simulink model "s_b4a4x32kf_54"  (R2018a)
settings: Solver=VariableStepDiscrete  StartTime=0.0  StopTime=10000  RelTol=1e-3
undefined symbols (not defined in the file): fft_stages, n_bits_ants, n_bits_xengs
libraries: xbsIndex_r4 x21235, casper_library_misc x37, casper_library_scopes x13, casper_library_delays x8, xbsReplacements_r4 x6, xps_library x4
(part 160 of 274)

== system s_b4a4x32kf_54/sys2/bf_pack_out0/Subsystem3/pipeline55 ==
  d : Inport
  Register0 : xbsIndex_r4/Register  init=0  rst=off  en=off  dbl_ovrd=off  block_type=register
      settings: SourceProductName=The database /home/jmanley/.matlab/R2018a/slblocks_master.db is locked, or a table in the database is locked. (database is locked)  block_version=11.4
  Register1 : xbsIndex_r4/Register  init=0  rst=off  en=off  dbl_ovrd=off  block_type=register
      settings: SourceProductName=The database /home/jmanley/.matlab/R2018a/slblocks_master.db is locked, or a table in the database is locked. (database is locked)  block_version=11.4
  q : Outport
  wires:
  Register0/1 -> Register1/1
  d/1 -> Register0/1
  Register1/1 -> q/1

== system s_b4a4x32kf_54/sys2/bf_pack_out0/Subsystem3/pipeline7 ==
  d : Inport
  Register0 : xbsIndex_r4/Register  init=0  rst=off  en=off  dbl_ovrd=off  block_type=register
      settings: SourceProductName=The database /home/jmanley/.matlab/R2018a/slblocks_master.db is locked, or a table in the database is locked. (database is locked)  block_version=11.4
  Register1 : xbsIndex_r4/Register  init=0  rst=off  en=off  dbl_ovrd=off  block_type=register
      settings: SourceProductName=The database /home/jmanley/.matlab/R2018a/slblocks_master.db is locked, or a table in the database is locked. (database is locked)  block_version=11.4
  q : Outport
  wires:
  Register0/1 -> Register1/1
  d/1 -> Register0/1
  Register1/1 -> q/1

== system s_b4a4x32kf_54/sys2/bf_pack_out0/data_fifo/bus_replicate ==
  in : Inport
  bussify : Subsystem  AncestorBlock=casper_library_flow_control/bus_create  mask(bus_create){inputNum=16}
      mask prompts: inputNum "Number of inputs:"
      mask init:
      | bus_create_init(gcb,...
      |     'inputNum', inputNum);
  out : Outport
  wires:
  in/1 -> bussify/1(in1), bussify/2(in2), bussify/3(in3), bussify/4(in4), bussify/5(in5), bussify/6(in6), bussify/7(in7), bussify/8(in8), bussify/9(in9), bussify/10(in10), bussify/11(in11), bussify/12(in12), bussify/13(in13), bussify/14(in14), bussify/15(in15), bussify/16(in16)
  bussify/1(bus_out) -> out/1

== system s_b4a4x32kf_54/sys2/bf_pack_out0/data_fifo/edge_detect ==
  in : Inport
  Delay : xbsIndex_r4/Delay  rst=off  infoeditControl=Selection of Reset will increase slice count due to use of real FFs and instead of SRLs  en=off  latency=1  reg_retiming=off  dbl_ovrd=off  block_type=delay
      settings: SourceProductName=The database /home/jmanley/.matlab/R2018a/slblocks_master.db is locked, or a table in the database is locked. (database is locked)  xl_area=[0, 0, 0, 0, 0, 0, 0]
  Inverter : xbsIndex_r4/Inverter  en=off  latency=0  dbl_ovrd=off  block_type=inv
      settings: SourceProductName=The database /home/jmanley/.matlab/R2018a/slblocks_master.db is locked, or a table in the database is locked. (database is locked)  xl_area=[0, 0, 0, 0, 0, 0, 0]
  edge_op : xbsIndex_r4/Logical  logical_function=AND  inputs=2  en=off  latency=0  precision=Full  arith_type=Unsigned  n_bits=8  bin_pt=2  align_bp=on  dbl_ovrd=off  block_type=logical
      settings: SourceProductName=The database /home/jmanley/.matlab/R2018a/slblocks_master.db is locked, or a table in the database is locked. (database is locked)  xl_area=[0, 0, 0, 0, 0, 0, 0]
  out : Outport
  wires:
  Inverter/1 -> edge_op/1
  edge_op/1 -> out/1
  in/1 -> Inverter/1, Delay/1
  Delay/1 -> edge_op/2

== system s_b4a4x32kf_54/sys2/bf_pack_out0/data_fifo/edge_detect1 ==
  in : Inport
  Delay : xbsIndex_r4/Delay  rst=off  infoeditControl=Selection of Reset will increase slice count due to use of real FFs and instead of SRLs  en=off  latency=1  reg_retiming=off  dbl_ovrd=off  block_type=delay
      settings: SourceProductName=The database /home/jmanley/.matlab/R2018a/slblocks_master.db is locked, or a table in the database is locked. (database is locked)  xl_area=[0, 0, 0, 0, 0, 0, 0]
  Inverter : xbsIndex_r4/Inverter  en=off  latency=0  dbl_ovrd=off  block_type=inv
      settings: SourceProductName=The database /home/jmanley/.matlab/R2018a/slblocks_master.db is locked, or a table in the database is locked. (database is locked)  xl_area=[0, 0, 0, 0, 0, 0, 0]
  edge_op : xbsIndex_r4/Logical  logical_function=AND  inputs=2  en=off  latency=0  precision=Full  arith_type=Unsigned  n_bits=8  bin_pt=2  align_bp=on  dbl_ovrd=off  block_type=logical
      settings: SourceProductName=The database /home/jmanley/.matlab/R2018a/slblocks_master.db is locked, or a table in the database is locked. (database is locked)  xl_area=[0, 0, 0, 0, 0, 0, 0]
  out : Outport
  wires:
  Inverter/1 -> edge_op/1
  edge_op/1 -> out/1
  in/1 -> Inverter/1, Delay/1
  Delay/1 -> edge_op/2

== system s_b4a4x32kf_54/sys2/bf_pack_out0/data_fifo/munge ==
  din : Inport
  join : Subsystem  AncestorBlock=casper_library_flow_control/bus_create  mask(bus_create){inputNum=16}
      mask prompts: inputNum "Number of inputs:"
      mask init:
      | bus_create_init(gcb,...
      |     'inputNum', inputNum);
  reinterpret : xbsIndex_r4/Reinterpret  force_arith_type=on  arith_type=Unsigned  force_bin_pt=on  bin_pt=0  block_type=reinterpret
      settings: SourceProductName=The database /home/jmanley/.matlab/R2018a/slblocks_master.db is locked, or a table in the database is locked. (database is locked)
  reinterpret_out : xbsIndex_r4/Reinterpret  force_arith_type=on  arith_type=Unsigned  force_bin_pt=on  bin_pt=0  block_type=reinterpret
      settings: SourceProductName=The database /home/jmanley/.matlab/R2018a/slblocks_master.db is locked, or a table in the database is locked. (database is locked)
  split : Subsystem  AncestorBlock=casper_library_flow_control/bus_expand  mask(bus_expand){mode=divisions of arbitrary size, outputNum=1, outputWidth=[16 16 16 16 16 16 16 16 16 16 16 16 16 16 16 16], outputBinaryPt=[0 0 0 0 0 0 0 0 0 0 0 0 0 0 0 0], outputArithmeticType=[0 0 0 0 0 0 0 0 0 0 0 0 0 0 0 0], show_format=off, outputToWorkspace=off, variablePrefix=out, outputToModelAsWell=on}
      mask prompts: outputNum "Number of outputs:"; outputWidth "Output width [msb ... lsb]:"; outputBinaryPt "Output binary point position [msb ... lsb]:"; outputArithmeticType "Output arithmetic type (ufix=0, fix=1, bool=2) [msb ... lsb]:"; show_format "Print format string?"; outputToWorkspace "Output to workspace?"; variablePrefix "Variable name prefix:"; outputToModelAsWell "Output to model as well?"
      mask help:
      | Expands a 'bus' made using a bus_create or Xilinx
      | concat block.
      | The input will be divided into the specified number
      | of outputs with the specified arithmetic types.
      | Divisions are made from most significant bit.
      mask init: same as s_b4a4x32kf_54/bus_expand
      settings: AttributesFormatString=16 outputs
      mask TypeOptions mode: divisions of equal size | divisions of arbitrary size
      mask Callback mode: bus_expand_callback();
      mask Callback outputWidth: bus_expand_callback();
      mask Callback outputToWorkspace: bus_expand_callback();
  dout : Outport
  wires:
  reinterpret_out/1 -> dout/1
  din/1 -> reinterpret/1
  reinterpret/1 -> split/1(bus_in)
  join/1(bus_out) -> reinterpret_out/1
  split/16(lsb_out1) -> join/1(in1)
  split/15(out2) -> join/2(in2)
  split/14(out3) -> join/3(in3)
  split/13(out4) -> join/4(in4)
  split/12(out5) -> join/5(in5)
  split/11(out6) -> join/6(in6)
  split/10(out7) -> join/7(in7)
  split/9(out8) -> join/8(in8)
  split/8(out9) -> join/9(in9)
  split/7(out10) -> join/10(in10)
  split/6(out11) -> join/11(in11)
  split/5(out12) -> join/12(in12)
  split/4(out13) -> join/13(in13)
  split/3(out14) -> join/14(in14)
  split/2(out15) -> join/15(in15)
  split/1(msb_out16) -> join/16(in16)

== system s_b4a4x32kf_54/sys2/bf_pack_out0/pack/edge_detect1 ==
  in : Inport
  Delay : xbsIndex_r4/Delay  rst=off  infoeditControl=Selection of Reset will increase slice count due to use of real FFs and instead of SRLs  en=off  latency=1  reg_retiming=off  dbl_ovrd=off  block_type=delay
      settings: SourceProductName=The database /home/jmanley/.matlab/R2018a/slblocks_master.db is locked, or a table in the database is locked. (database is locked)  xl_area=[0, 0, 0, 0, 0, 0, 0]
  Inverter : xbsIndex_r4/Inverter  en=off  latency=0  dbl_ovrd=off  block_type=inv
      settings: SourceProductName=The database /home/jmanley/.matlab/R2018a/slblocks_master.db is locked, or a table in the database is locked. (database is locked)  xl_area=[0, 0, 0, 0, 0, 0, 0]
  edge_op : xbsIndex_r4/Logical  logical_function=AND  inputs=2  en=off  latency=0  precision=Full  arith_type=Unsigned  n_bits=8  bin_pt=2  align_bp=on  dbl_ovrd=off  block_type=logical
      settings: SourceProductName=The database /home/jmanley/.matlab/R2018a/slblocks_master.db is locked, or a table in the database is locked. (database is locked)  xl_area=[0, 0, 0, 0, 0, 0, 0]
  out : Outport
  wires:
  Inverter/1 -> edge_op/1
  edge_op/1 -> out/1
  in/1 -> Inverter/1, Delay/1
  Delay/1 -> edge_op/2

== system s_b4a4x32kf_54/sys2/bf_pack_out0/pack/edge_detect3 ==
  in : Inport
  Delay : xbsIndex_r4/Delay  rst=off  infoeditControl=Selection of Reset will increase slice count due to use of real FFs and instead of SRLs  en=off  latency=1  reg_retiming=off  dbl_ovrd=off  block_type=delay
      settings: SourceProductName=The database /home/jmanley/.matlab/R2018a/slblocks_master.db is locked, or a table in the database is locked. (database is locked)  xl_area=[0, 0, 0, 0, 0, 0, 0]
  Inverter : xbsIndex_r4/Inverter  en=off  latency=0  dbl_ovrd=off  block_type=inv
      settings: SourceProductName=The database /home/jmanley/.matlab/R2018a/slblocks_master.db is locked, or a table in the database is locked. (database is locked)  xl_area=[0, 0, 0, 0, 0, 0, 0]
  edge_op : xbsIndex_r4/Logical  logical_function=NOR  inputs=2  en=off  latency=0  precision=Full  arith_type=Unsigned  n_bits=8  bin_pt=2  align_bp=on  dbl_ovrd=off  block_type=logical
      settings: SourceProductName=The database /home/jmanley/.matlab/R2018a/slblocks_master.db is locked, or a table in the database is locked. (database is locked)  xl_area=[0, 0, 0, 0, 0, 0, 0]
  out : Outport
  wires:
  Inverter/1 -> edge_op/1
  edge_op/1 -> out/1
  in/1 -> Inverter/1, Delay/1
  Delay/1 -> edge_op/2

== system s_b4a4x32kf_54/sys2/bf_pack_out1/Subsystem3/edge_detect ==
  in : Inport
  Delay : xbsIndex_r4/Delay  rst=off  infoeditControl=Selection of Reset will increase slice count due to use of real FFs and instead of SRLs  en=off  latency=1  reg_retiming=off  dbl_ovrd=off  block_type=delay
      settings: SourceProductName=The database /home/jmanley/.matlab/R2018a/slblocks_master.db is locked, or a table in the database is locked. (database is locked)  xl_area=[0, 0, 0, 0, 0, 0, 0]
  Inverter : xbsIndex_r4/Inverter  en=off  latency=0  dbl_ovrd=off  block_type=inv
      settings: SourceProductName=The database /home/jmanley/.matlab/R2018a/slblocks_master.db is locked, or a table in the database is locked. (database is locked)  xl_area=[0, 0, 0, 0, 0, 0, 0]
  edge_op : xbsIndex_r4/Logical  logical_function=NOR  inputs=2  en=off  latency=0  precision=Full  arith_type=Unsigned  n_bits=8  bin_pt=2  align_bp=on  dbl_ovrd=off  block_type=logical
      settings: SourceProductName=The database /home/jmanley/.matlab/R2018a/slblocks_master.db is locked, or a table in the database is locked. (database is locked)  xl_area=[0, 0, 0, 0, 0, 0, 0]
  out : Outport
  wires:
  Inverter/1 -> edge_op/1
  edge_op/1 -> out/1
  in/1 -> Inverter/1, Delay/1
  Delay/1 -> edge_op/2

== system s_b4a4x32kf_54/sys2/bf_pack_out1/Subsystem3/edge_detect1 ==
  in : Inport
  Delay : xbsIndex_r4/Delay  rst=off  infoeditControl=Selection of Reset will increase slice count due to use of real FFs and instead of SRLs  en=off  latency=1  reg_retiming=off  dbl_ovrd=off  block_type=delay
      settings: SourceProductName=The database /home/jmanley/.matlab/R2018a/slblocks_master.db is locked, or a table in the database is locked. (database is locked)  xl_area=[0, 0, 0, 0, 0, 0, 0]
  Inverter : xbsIndex_r4/Inverter  en=off  latency=0  dbl_ovrd=off  block_type=inv
      settings: SourceProductName=The database /home/jmanley/.matlab/R2018a/slblocks_master.db is locked, or a table in the database is locked. (database is locked)  xl_area=[0, 0, 0, 0, 0, 0, 0]
  edge_op : xbsIndex_r4/Logical  logical_function=NOR  inputs=2  en=off  latency=0  precision=Full  arith_type=Unsigned  n_bits=8  bin_pt=2  align_bp=on  dbl_ovrd=off  block_type=logical
      settings: SourceProductName=The database /home/jmanley/.matlab/R2018a/slblocks_master.db is locked, or a table in the database is locked. (database is locked)  xl_area=[0, 0, 0, 0, 0, 0, 0]
  out : Outport
  wires:
  Inverter/1 -> edge_op/1
  edge_op/1 -> out/1
  in/1 -> Inverter/1, Delay/1
  Delay/1 -> edge_op/2

== system s_b4a4x32kf_54/sys2/bf_pack_out1/Subsystem3/pipeline1 ==
  d : Inport
  Register0 : xbsIndex_r4/Register  init=0  rst=off  en=off  dbl_ovrd=off  block_type=register
      settings: SourceProductName=The database /home/jmanley/.matlab/R2018a/slblocks_master.db is locked, or a table in the database is locked. (database is locked)  block_version=11.4
  Register1 : xbsIndex_r4/Register  init=0  rst=off  en=off  dbl_ovrd=off  block_type=register
      settings: SourceProductName=The database /home/jmanley/.matlab/R2018a/slblocks_master.db is locked, or a table in the database is locked. (database is locked)  block_version=11.4
  q : Outport
  wires:
  Register0/1 -> Register1/1
  d/1 -> Register0/1
  Register1/1 -> q/1

== system s_b4a4x32kf_54/sys2/bf_pack_out1/Subsystem3/pipeline2 ==
  d : Inport
  Register0 : xbsIndex_r4/Register  init=0  rst=off  en=off  dbl_ovrd=off  block_type=register
      settings: SourceProductName=The database /home/jmanley/.matlab/R2018a/slblocks_master.db is locked, or a table in the database is locked. (database is locked)  block_version=11.4
  Register1 : xbsIndex_r4/Register  init=0  rst=off  en=off  dbl_ovrd=off  block_type=register
      settings: SourceProductName=The database /home/jmanley/.matlab/R2018a/slblocks_master.db is locked, or a table in the database is locked. (database is locked)  block_version=11.4
  q : Outport
  wires:
  Register0/1 -> Register1/1
  d/1 -> Register0/1
  Register1/1 -> q/1

== system s_b4a4x32kf_54/sys2/bf_pack_out1/Subsystem3/pipeline53 ==
  d : Inport
  Register0 : xbsIndex_r4/Register  init=0  rst=off  en=off  dbl_ovrd=off  block_type=register
      settings: SourceProductName=The database /home/jmanley/.matlab/R2018a/slblocks_master.db is locked, or a table in the database is locked. (database is locked)  block_version=11.4
  Register1 : xbsIndex_r4/Register  init=0  rst=off  en=off  dbl_ovrd=off  block_type=register
      settings: SourceProductName=The database /home/jmanley/.matlab/R2018a/slblocks_master.db is locked, or a table in the database is locked. (database is locked)  block_version=11.4
  q : Outport
  wires:
  Register0/1 -> Register1/1
  d/1 -> Register0/1
  Register1/1 -> q/1

== system s_b4a4x32kf_54/sys2/bf_pack_out1/Subsystem3/pipeline54 ==
  d : Inport
  Register0 : xbsIndex_r4/Register  init=0  rst=off  en=off  dbl_ovrd=off  block_type=register
      settings: SourceProductName=The database /home/jmanley/.matlab/R2018a/slblocks_master.db is locked, or a table in the database is locked. (database is locked)  block_version=11.4
  Register1 : xbsIndex_r4/Register  init=0  rst=off  en=off  dbl_ovrd=off  block_type=register
      settings: SourceProductName=The database /home/jmanley/.matlab/R2018a/slblocks_master.db is locked, or a table in the database is locked. (database is locked)  block_version=11.4
  q : Outport
  wires:
  Register0/1 -> Register1/1
  d/1 -> Register0/1
  Register1/1 -> q/1

== system s_b4a4x32kf_54/sys2/bf_pack_out1/Subsystem3/pipeline55 ==
  d : Inport
  Register0 : xbsIndex_r4/Register  init=0  rst=off  en=off  dbl_ovrd=off  block_type=register
      settings: SourceProductName=The database /home/jmanley/.matlab/R2018a/slblocks_master.db is locked, or a table in the database is locked. (database is locked)  block_version=11.4
  Register1 : xbsIndex_r4/Register  init=0  rst=off  en=off  dbl_ovrd=off  block_type=register
      settings: SourceProductName=The database /home/jmanley/.matlab/R2018a/slblocks_master.db is locked, or a table in the database is locked. (database is locked)  block_version=11.4
  q : Outport
  wires:
  Register0/1 -> Register1/1
  d/1 -> Register0/1
  Register1/1 -> q/1

== system s_b4a4x32kf_54/sys2/bf_pack_out1/Subsystem3/pipeline7 ==
  d : Inport
  Register0 : xbsIndex_r4/Register  init=0  rst=off  en=off  dbl_ovrd=off  block_type=register
      settings: SourceProductName=The database /home/jmanley/.matlab/R2018a/slblocks_master.db is locked, or a table in the database is locked. (database is locked)  block_version=11.4
  Register1 : xbsIndex_r4/Register  init=0  rst=off  en=off  dbl_ovrd=off  block_type=register
      settings: SourceProductName=The database /home/jmanley/.matlab/R2018a/slblocks_master.db is locked, or a table in the database is locked. (database is locked)  block_version=11.4
  q : Outport
  wires:
  Register0/1 -> Register1/1
  d/1 -> Register0/1
  Register1/1 -> q/1

== system s_b4a4x32kf_54/sys2/bf_pack_out1/data_fifo/bus_replicate ==
  in : Inport
  bussify : Subsystem  AncestorBlock=casper_library_flow_control/bus_create  mask(bus_create){inputNum=16}
      mask prompts: inputNum "Number of inputs:"
      mask init:
      | bus_create_init(gcb,...
      |     'inputNum', inputNum);
  out : Outport
  wires:
  in/1 -> bussify/1(in1), bussify/2(in2), bussify/3(in3), bussify/4(in4), bussify/5(in5), bussify/6(in6), bussify/7(in7), bussify/8(in8), bussify/9(in9), bussify/10(in10), bussify/11(in11), bussify/12(in12), bussify/13(in13), bussify/14(in14), bussify/15(in15), bussify/16(in16)
  bussify/1(bus_out) -> out/1

== system s_b4a4x32kf_54/sys2/bf_pack_out1/data_fifo/edge_detect ==
  in : Inport
  Delay : xbsIndex_r4/Delay  rst=off  infoeditControl=Selection of Reset will increase slice count due to use of real FFs and instead of SRLs  en=off  latency=1  reg_retiming=off  dbl_ovrd=off  block_type=delay
      settings: SourceProductName=The database /home/jmanley/.matlab/R2018a/slblocks_master.db is locked, or a table in the database is locked. (database is locked)  xl_area=[0, 0, 0, 0, 0, 0, 0]
  Inverter : xbsIndex_r4/Inverter  en=off  latency=0  dbl_ovrd=off  block_type=inv
      settings: SourceProductName=The database /home/jmanley/.matlab/R2018a/slblocks_master.db is locked, or a table in the database is locked. (database is locked)  xl_area=[0, 0, 0, 0, 0, 0, 0]
  edge_op : xbsIndex_r4/Logical  logical_function=AND  inputs=2  en=off  latency=0  precision=Full  arith_type=Unsigned  n_bits=8  bin_pt=2  align_bp=on  dbl_ovrd=off  block_type=logical
      settings: SourceProductName=The database /home/jmanley/.matlab/R2018a/slblocks_master.db is locked, or a table in the database is locked. (database is locked)  xl_area=[0, 0, 0, 0, 0, 0, 0]
  out : Outport
  wires:
  Inverter/1 -> edge_op/1
  edge_op/1 -> out/1
  in/1 -> Inverter/1, Delay/1
  Delay/1 -> edge_op/2

== system s_b4a4x32kf_54/sys2/bf_pack_out1/data_fifo/edge_detect1 ==
  in : Inport
  Delay : xbsIndex_r4/Delay  rst=off  infoeditControl=Selection of Reset will increase slice count due to use of real FFs and instead of SRLs  en=off  latency=1  reg_retiming=off  dbl_ovrd=off  block_type=delay
      settings: SourceProductName=The database /home/jmanley/.matlab/R2018a/slblocks_master.db is locked, or a table in the database is locked. (database is locked)  xl_area=[0, 0, 0, 0, 0, 0, 0]
  Inverter : xbsIndex_r4/Inverter  en=off  latency=0  dbl_ovrd=off  block_type=inv
      settings: SourceProductName=The database /home/jmanley/.matlab/R2018a/slblocks_master.db is locked, or a table in the database is locked. (database is locked)  xl_area=[0, 0, 0, 0, 0, 0, 0]
  edge_op : xbsIndex_r4/Logical  logical_function=AND  inputs=2  en=off  latency=0  precision=Full  arith_type=Unsigned  n_bits=8  bin_pt=2  align_bp=on  dbl_ovrd=off  block_type=logical
      settings: SourceProductName=The database /home/jmanley/.matlab/R2018a/slblocks_master.db is locked, or a table in the database is locked. (database is locked)  xl_area=[0, 0, 0, 0, 0, 0, 0]
  out : Outport
  wires:
  Inverter/1 -> edge_op/1
  edge_op/1 -> out/1
  in/1 -> Inverter/1, Delay/1
  Delay/1 -> edge_op/2

== system s_b4a4x32kf_54/sys2/bf_pack_out1/data_fifo/munge ==
  din : Inport
  join : Subsystem  AncestorBlock=casper_library_flow_control/bus_create  mask(bus_create){inputNum=16}
      mask prompts: inputNum "Number of inputs:"
      mask init:
      | bus_create_init(gcb,...
      |     'inputNum', inputNum);
  reinterpret : xbsIndex_r4/Reinterpret  force_arith_type=on  arith_type=Unsigned  force_bin_pt=on  bin_pt=0  block_type=reinterpret
      settings: SourceProductName=The database /home/jmanley/.matlab/R2018a/slblocks_master.db is locked, or a table in the database is locked. (database is locked)
  reinterpret_out : xbsIndex_r4/Reinterpret  force_arith_type=on  arith_type=Unsigned  force_bin_pt=on  bin_pt=0  block_type=reinterpret
      settings: SourceProductName=The database /home/jmanley/.matlab/R2018a/slblocks_master.db is locked, or a table in the database is locked. (database is locked)
  split : Subsystem  AncestorBlock=casper_library_flow_control/bus_expand  mask(bus_expand){mode=divisions of arbitrary size, outputNum=1, outputWidth=[16 16 16 16 16 16 16 16 16 16 16 16 16 16 16 16], outputBinaryPt=[0 0 0 0 0 0 0 0 0 0 0 0 0 0 0 0], outputArithmeticType=[0 0 0 0 0 0 0 0 0 0 0 0 0 0 0 0], show_format=off, outputToWorkspace=off, variablePrefix=out, outputToModelAsWell=on}
      mask prompts: outputNum "Number of outputs:"; outputWidth "Output width [msb ... lsb]:"; outputBinaryPt "Output binary point position [msb ... lsb]:"; outputArithmeticType "Output arithmetic type (ufix=0, fix=1, bool=2) [msb ... lsb]:"; show_format "Print format string?"; outputToWorkspace "Output to workspace?"; variablePrefix "Variable name prefix:"; outputToModelAsWell "Output to model as well?"
      mask help:
      | Expands a 'bus' made using a bus_create or Xilinx
      | concat block.
      | The input will be divided into the specified number
      | of outputs with the specified arithmetic types.
      | Divisions are made from most significant bit.
      mask init: same as s_b4a4x32kf_54/bus_expand
      settings: AttributesFormatString=16 outputs
      mask TypeOptions mode: divisions of equal size | divisions of arbitrary size
      mask Callback mode: bus_expand_callback();
      mask Callback outputWidth: bus_expand_callback();
      mask Callback outputToWorkspace: bus_expand_callback();
  dout : Outport
  wires:
  reinterpret_out/1 -> dout/1
  din/1 -> reinterpret/1
  reinterpret/1 -> split/1(bus_in)
  join/1(bus_out) -> reinterpret_out/1
  split/16(lsb_out1) -> join/1(in1)
  split/15(out2) -> join/2(in2)
  split/14(out3) -> join/3(in3)
  split/13(out4) -> join/4(in4)
  split/12(out5) -> join/5(in5)
  split/11(out6) -> join/6(in6)
  split/10(out7) -> join/7(in7)
  split/9(out8) -> join/8(in8)
  split/8(out9) -> join/9(in9)
  split/7(out10) -> join/10(in10)
  split/6(out11) -> join/11(in11)
  split/5(out12) -> join/12(in12)
  split/4(out13) -> join/13(in13)
  split/3(out14) -> join/14(in14)
  split/2(out15) -> join/15(in15)
  split/1(msb_out16) -> join/16(in16)

== system s_b4a4x32kf_54/sys2/bf_pack_out1/pack/edge_detect1 ==
  in : Inport
  Delay : xbsIndex_r4/Delay  rst=off  infoeditControl=Selection of Reset will increase slice count due to use of real FFs and instead of SRLs  en=off  latency=1  reg_retiming=off  dbl_ovrd=off  block_type=delay
      settings: SourceProductName=The database /home/jmanley/.matlab/R2018a/slblocks_master.db is locked, or a table in the database is locked. (database is locked)  xl_area=[0, 0, 0, 0, 0, 0, 0]
  Inverter : xbsIndex_r4/Inverter  en=off  latency=0  dbl_ovrd=off  block_type=inv
      settings: SourceProductName=The database /home/jmanley/.matlab/R2018a/slblocks_master.db is locked, or a table in the database is locked. (database is locked)  xl_area=[0, 0, 0, 0, 0, 0, 0]
  edge_op : xbsIndex_r4/Logical  logical_function=AND  inputs=2  en=off  latency=0  precision=Full  arith_type=Unsigned  n_bits=8  bin_pt=2  align_bp=on  dbl_ovrd=off  block_type=logical
      settings: SourceProductName=The database /home/jmanley/.matlab/R2018a/slblocks_master.db is locked, or a table in the database is locked. (database is locked)  xl_area=[0, 0, 0, 0, 0, 0, 0]
  out : Outport
  wires:
  Inverter/1 -> edge_op/1
  edge_op/1 -> out/1
  in/1 -> Inverter/1, Delay/1
  Delay/1 -> edge_op/2

== system s_b4a4x32kf_54/sys2/bf_pack_out1/pack/edge_detect3 ==
  in : Inport
  Delay : xbsIndex_r4/Delay  rst=off  infoeditControl=Selection of Reset will increase slice count due to use of real FFs and instead of SRLs  en=off  latency=1  reg_retiming=off  dbl_ovrd=off  block_type=delay
      settings: SourceProductName=The database /home/jmanley/.matlab/R2018a/slblocks_master.db is locked, or a table in the database is locked. (database is locked)  xl_area=[0, 0, 0, 0, 0, 0, 0]
  Inverter : xbsIndex_r4/Inverter  en=off  latency=0  dbl_ovrd=off  block_type=inv
      settings: SourceProductName=The database /home/jmanley/.matlab/R2018a/slblocks_master.db is locked, or a table in the database is locked. (database is locked)  xl_area=[0, 0, 0, 0, 0, 0, 0]
  edge_op : xbsIndex_r4/Logical  logical_function=NOR  inputs=2  en=off  latency=0  precision=Full  arith_type=Unsigned  n_bits=8  bin_pt=2  align_bp=on  dbl_ovrd=off  block_type=logical
      settings: SourceProductName=The database /home/jmanley/.matlab/R2018a/slblocks_master.db is locked, or a table in the database is locked. (database is locked)  xl_area=[0, 0, 0, 0, 0, 0, 0]
  out : Outport
  wires:
  Inverter/1 -> edge_op/1
  edge_op/1 -> out/1
  in/1 -> Inverter/1, Delay/1
  Delay/1 -> edge_op/2

== system s_b4a4x32kf_54/sys2/pkt_reord/bus_replicate/bussify ==
  in1 : Inport
  reinterpret1 : xbsIndex_r4/Reinterpret  force_arith_type=on  arith_type=Unsigned  force_bin_pt=on  bin_pt=0  block_type=reinterpret
      settings: SourceProductName=The database /home/jmanley/.matlab/R2018a/slblocks_master.db is locked, or a table in the database is locked. (database is locked)  infoedit="Changes signal type without altering the binary representation.   You can changed the signal between signed and unsigned, and relocate the binary point.<br><br>Hardware notes: In hardware this block costs nothing.<br><br>Example:  Suppose the input is 6 bits wide, signed, with 2 fractional bits, and the output is forced to unsigned with 0 fractional bits.  Then an input of -2.0 (1110.00 in binary 2's complement) becomes an output of 56 (111000 in binary)."
  bus_out : Outport
  wires:
  in1/1 -> reinterpret1/1
  reinterpret1/1 -> bus_out/1

== system s_b4a4x32kf_54/sys2/pkt_reord/input_control/adder_tree ==
  sync : Inport
  din1 : Inport  Port=2
  din2 : Inport  Port=3
  din3 : Inport  Port=4
  addr1 : xbsIndex_r4/AddSub  mode=Addition  use_carryin=off  use_carryout=off  en=off  latency=2  precision=Full  arith_type=Unsigned  n_bits=16  bin_pt=14  quantization=Truncate  overflow=Wrap  use_behavioral_HDL=off  hw_selection=Fabric  pipelined=on  use_rpm=on  dbl_ovrd=off  block_type=addsub
      settings: SourceProductName=The database /home/jmanley/.matlab/R2018a/slblocks_master.db is locked, or a table in the database is locked. (database is locked)
  addr3 : xbsIndex_r4/AddSub  mode=Addition  use_carryin=off  use_carryout=off  en=off  latency=2  precision=Full  arith_type=Unsigned  n_bits=16  bin_pt=14  quantization=Truncate  overflow=Wrap  use_behavioral_HDL=off  hw_selection=Fabric  pipelined=on  use_rpm=on  dbl_ovrd=off  block_type=addsub
      settings: SourceProductName=The database /home/jmanley/.matlab/R2018a/slblocks_master.db is locked, or a table in the database is locked. (database is locked)
  dly2 : xbsIndex_r4/Delay  rst=off  infoeditControl=Selection of Reset will increase slice count due to use of real FFs and instead of SRLs  en=off  latency=2  reg_retiming=on  dbl_ovrd=off  block_type=delay
      settings: SourceProductName=The database /home/jmanley/.matlab/R2018a/slblocks_master.db is locked, or a table in the database is locked. (database is locked)
  sync_delay : xbsIndex_r4/Delay  rst=off  infoeditControl=Selection of Reset will increase slice count due to use of real FFs and instead of SRLs  en=off  latency=4  reg_retiming=on  dbl_ovrd=off  block_type=delay
      settings: SourceProductName=The database /home/jmanley/.matlab/R2018a/slblocks_master.db is locked, or a table in the database is locked. (database is locked)  block_version=11.4
  sync_out : Outport
  dout : Outport  Port=2
  wires:
  sync/1 -> sync_delay/1
  sync_delay/1 -> sync_out/1
  din1/1 -> addr1/1
  din2/1 -> addr1/2
  din3/1 -> dly2/1
  addr1/1 -> addr3/1
  dly2/1 -> addr3/2
  addr3/1 -> dout/1

== system s_b4a4x32kf_54/sys2/pkt_reord/input_control/mcnt_thresh ==
  note: we record if this is the first timestamp.
      | If it is we capture it even if out of bounds
  note: capture any new mcnts which
      | are within (1/2 buffer - 1)
      | of the previous mcnt.
      | This prevents locking onto
      | bad mcnts
  note: timeout of a bad
      | master count
      | in ~2^20 clocks
  mcnt : Inport
  en : Inport  Port=2
  AddSub : xbsIndex_r4/AddSub  mode=Addition  use_carryin=off  use_carryout=off  en=off  latency=2  precision=User Defined  arith_type=Unsigned  n_bits=n_bits_timestamp + (chan_bits-xeng_bits)  bin_pt=0  quantization=Truncate  overflow=Wrap  use_behavioral_HDL=on  hw_selection=Fabric  pipelined=off  dbl_ovrd=off  block_type=addsub
      settings: SourceProductName=The database /home/jmanley/.matlab/R2018a/slblocks_master.db is locked, or a table in the database is locked. (database is locked)
  Constant1 : xbsIndex_r4/Constant  const=(2^(window_bits - 2)) + 1  gui_display_data_type=Fixed-point  arith_type=Unsigned  n_bits=window_bits  bin_pt=0  preci_type=Single  exp_width=8  frac_width=24  explicit_period=on  period=1  equ=P=C  opselect=C  inp2=PCIN>>17  opr=+  inp1=P  carry=CIN  dbl_ovrd=off  block_type=constant
      settings: SourceProductName=The database /home/jmanley/.matlab/R2018a/slblocks_master.db is locked, or a table in the database is locked. (database is locked)
  Counter : xbsIndex_r4/Counter  cnt_type=Free Running  cnt_to=Inf  operation=Up  start_count=0  cnt_by_val=1  arith_type=Unsigned  n_bits=21  bin_pt=0  load_pin=off  rst=on  en=off  explicit_period=on  period=1  use_behavioral_HDL=off  implementation=Fabric  use_rpm=on  dbl_ovrd=off  block_type=counter
      settings: SourceProductName=The database /home/jmanley/.matlab/R2018a/slblocks_master.db is locked, or a table in the database is locked. (database is locked)  xl_area=[0, 0, 0, 0, 0, 0, 0]
  Delay : xbsIndex_r4/Delay  rst=off  infoeditControl=Selection of Reset will increase slice count due to use of real FFs and instead of SRLs  en=off  latency=2  reg_retiming=on  dbl_ovrd=off  block_type=delay
      settings: SourceProductName=The database /home/jmanley/.matlab/R2018a/slblocks_master.db is locked, or a table in the database is locked. (database is locked)  xl_area=[0, 0, 0, 0, 0, 0, 0]
  Delay1 : xbsIndex_r4/Delay  rst=off  infoeditControl=Selection of Reset will increase slice count due to use of real FFs and instead of SRLs  en=off  latency=1  reg_retiming=on  dbl_ovrd=off  block_type=delay
      settings: SourceProductName=The database /home/jmanley/.matlab/R2018a/slblocks_master.db is locked, or a table in the database is locked. (database is locked)  xl_area=[0, 0, 0, 0, 0, 0, 0]
  Gateway Out{,1..6} (7 alike) : xbsIndex_r4/Gateway Out  inherit_from_input=off  hdl_port=on  rows=1  columns=1  UseAsDAC=off  DACChannel='1'  interface=None  automatic_assignment=on  address_offset=hex2dec('00')  intf_name=''  intf_description=''  timing_constraint=None  locs_specified=off  LOCs={}  io_standard={}  block_type=gatewayout
      settings: SourceProductName=The database /home/jmanley/.matlab/R2018a/slblocks_master.db is locked, or a table in the database is locked. (database is locked)
  Inverter : xbsIndex_r4/Inverter  en=off  latency=0  dbl_ovrd=off  block_type=inv
      settings: SourceProductName=The database /home/jmanley/.matlab/R2018a/slblocks_master.db is locked, or a table in the database is locked. (database is locked)
  Logical : xbsIndex_r4/Logical  logical_function=AND  inputs=2  en=off  latency=0  precision=Full  arith_type=Unsigned  n_bits=8  bin_pt=2  align_bp=on  dbl_ovrd=off  block_type=logical
      settings: SourceProductName=The database /home/jmanley/.matlab/R2018a/slblocks_master.db is locked, or a table in the database is locked. (database is locked)  xl_area=[0, 0, 0, 0, 0, 0, 0]
  Logical1 : xbsIndex_r4/Logical  logical_function=OR  inputs=3  en=off  latency=0  precision=Full  arith_type=Unsigned  n_bits=8  bin_pt=2  align_bp=on  dbl_ovrd=off  block_type=logical
      settings: SourceProductName=The database /home/jmanley/.matlab/R2018a/slblocks_master.db is locked, or a table in the database is locked. (database is locked)  xl_area=[0, 0, 0, 0, 0, 0, 0]
  Register : xbsIndex_r4/Delay  rst=off  infoeditControl=Selection of Reset will increase slice count due to use of real FFs and instead of SRLs  en=on  latency=1  reg_retiming=on  dbl_ovrd=off  block_type=delay
      settings: SourceProductName=The database /home/jmanley/.matlab/R2018a/slblocks_master.db is locked, or a table in the database is locked. (database is locked)
  Relational : xbsIndex_r4/Relational  mode=a>b  op_type=Bool  en=off  latency=1  dbl_ovrd=off  block_type=relational
      settings: SourceProductName=The database /home/jmanley/.matlab/R2018a/slblocks_master.db is locked, or a table in the database is locked. (database is locked)  xl_area=[0, 0, 0, 0, 0, 0, 0]  block_version=10.1.3
  Relational1 : xbsIndex_r4/Relational  mode=a<=b  op_type=Bool  en=off  latency=1  dbl_ovrd=off  block_type=relational
      settings: SourceProductName=The database /home/jmanley/.matlab/R2018a/slblocks_master.db is locked, or a table in the database is locked. (database is locked)  xl_area=[0, 0, 0, 0, 0, 0, 0]  block_version=10.1.3
  Scope1 : Scope  NumInputPorts=7
  Slice : xbsIndex_r4/Slice  nbits=1  boolean_output=on  mode=Upper Bit Location + Width  bit1=0  base1=MSB of Input  bit0=0  base0=LSB of Input  dbl_ovrd=off  block_type=slice
      settings: SourceProductName=The database /home/jmanley/.matlab/R2018a/slblocks_master.db is locked, or a table in the database is locked. (database is locked)  infoedit="Extracts a given range of bits from each input sample and presents it at the output.  The output type is ordinarily unsigned with binary point at zero, but can be Boolean when the slice is one bit wide.<P><P>Hardware notes: In hardware this block costs nothing."  block_version=10.1.3
  edge_detect : Subsystem  mask(edge_detect){edge=Rising, polarity=Active High, x_in=[0 0.08 0.08 0.16 0.16 0.24 0.24 0.32 0.32 0.4], y_in=[-1 -1  1  1  1  1  1  1  1  1], x_out=[0.6 0.68 0.68 0.76 0.76 0.84 0.84 0.92 0.92 1], y_out=[-1 -1  1  1 -1 -1 -1 -1 -1 -1]}
      mask prompts: edge "Edge Type"; polarity "Output Polarity"; x_in "Input X Positions"; y_in "Input Y Positions"; x_out "Output X Positions"; y_out "Output Y Positions"
      mask help: Output is active for one-cycle after each edge of the specified type (i.e. rising, falling or both).
      mask init: same as s_b4a4x32kf_54/edge_detect
      settings: AttributesFormatString=|
      | rising edges
      | active high
      mask Help: Output is active for one-cycle after each edge of the specified type (i.e. rising, falling, or both).  Latency is zero.
      mask TypeOptions edge: Rising | Falling | Both
      mask TypeOptions polarity: Active High | Active Low
      mask Display:
      | plot(x_in_num,0.5+y_in_num*0.2);
      | plot(x_out_num,0.5+y_out_num*0.2);
  not_first : xbsIndex_r4/Delay  rst=off  infoeditControl=Selection of Reset will increase slice count due to use of real FFs and instead of SRLs  en=on  latency=1  reg_retiming=on  dbl_ovrd=off  block_type=delay
      settings: SourceProductName=The database /home/jmanley/.matlab/R2018a/slblocks_master.db is locked, or a table in the database is locked. (database is locked)
  maxcnt : Outport
  mcnt_timeout : Outport  Port=2
  wires:
  Relational1/1 -> Logical/2
  mcnt/1 -> Relational1/1, Relational/1, Gateway Out/1, Delay1/1
  Slice/1 -> edge_detect/1(in), Logical1/1
  Logical1/1 -> Counter/1, Register/2, Gateway Out4/1
  Logical/1 -> Logical1/2, Gateway Out2/1
  Counter/1 -> Gateway Out1/1, Slice/1
  Relational/1 -> Logical/1
  Register/1 -> AddSub/1, maxcnt/1, Gateway Out5/1, Delay/1
  AddSub/1 -> Gateway Out6/1, Relational1/2
  en/1 -> not_first/1, not_first/2
  Inverter/1 -> Gateway Out3/1, Logical1/3
  Delay1/1 -> Register/1
  Gateway Out/1 -> Scope1/1
  Gateway Out1/1 -> Scope1/2
  Gateway Out2/1 -> Scope1/3
  Gateway Out3/1 -> Scope1/4
  Gateway Out4/1 -> Scope1/5
  Gateway Out5/1 -> Scope1/6
  Gateway Out6/1 -> Scope1/7
  Delay/1 -> Relational/2
  not_first/1 -> Inverter/1
  Constant1/1 -> AddSub/2
  edge_detect/1(out) -> mcnt_timeout/1

== system s_b4a4x32kf_54/sys2/pkt_reord/munge/join ==
  in1 : Inport
  in2 : Inport  Port=2
  in3 : Inport  Port=3
  in4 : Inport  Port=4
  in5 : Inport  Port=5
  in6 : Inport  Port=6
  in7 : Inport  Port=7
  in8 : Inport  Port=8
  in9 : Inport  Port=9
  in10 : Inport  Port=10
  in11 : Inport  Port=11
  in12 : Inport  Port=12
  in13 : Inport  Port=13
  in14 : Inport  Port=14
  in15 : Inport  Port=15
  in16 : Inport  Port=16
  concatenate : xbsIndex_r4/Concat  num_inputs=16  dbl_ovrd=off  block_type=concat
      settings: SourceProductName=The database /home/jmanley/.matlab/R2018a/slblocks_master.db is locked, or a table in the database is locked. (database is locked)
  reinterpret{1..16} (16 alike) : xbsIndex_r4/Reinterpret  force_arith_type=on  arith_type=Unsigned  force_bin_pt=on  bin_pt=0  block_type=reinterpret
      reinterpret1 settings: SourceProductName=The database /home/jmanley/.matlab/R2018a/slblocks_master.db is locked, or a table in the database is locked. (database is locked)  infoedit="Changes signal type without altering the binary representation.   You can changed the signal between signed and unsigned, and relocate the binary point.<br><br>Hardware notes: In hardware this block costs nothing.<br><br>Example:  Suppose the input is 6 bits wide, signed, with 2 fractional bits, and the output is forced to unsigned with 0 fractional bits.  Then an input of -2.0 (1110.00 in binary 2's complement) becomes an output of 56 (111000 in binary)."
      reinterpret10 settings: SourceProductName=The database /home/jmanley/.matlab/R2018a/slblocks_master.db is locked, or a table in the database is locked. (database is locked)
      reinterpret11 settings: SourceProductName=The database /home/jmanley/.matlab/R2018a/slblocks_master.db is locked, or a table in the database is locked. (database is locked)
      reinterpret12 settings: SourceProductName=The database /home/jmanley/.matlab/R2018a/slblocks_master.db is locked, or a table in the database is locked. (database is locked)
      reinterpret13 settings: SourceProductName=The database /home/jmanley/.matlab/R2018a/slblocks_master.db is locked, or a table in the database is locked. (database is locked)
      reinterpret14 settings: SourceProductName=The database /home/jmanley/.matlab/R2018a/slblocks_master.db is locked, or a table in the database is locked. (database is locked)
      reinterpret15 settings: SourceProductName=The database /home/jmanley/.matlab/R2018a/slblocks_master.db is locked, or a table in the database is locked. (database is locked)
      reinterpret16 settings: SourceProductName=The database /home/jmanley/.matlab/R2018a/slblocks_master.db is locked, or a table in the database is locked. (database is locked)
      reinterpret2 settings: SourceProductName=The database /home/jmanley/.matlab/R2018a/slblocks_master.db is locked, or a table in the database is locked. (database is locked)  infoedit="Changes signal type without altering the binary representation.   You can changed the signal between signed and unsigned, and relocate the binary point.<br><br>Hardware notes: In hardware this block costs nothing.<br><br>Example:  Suppose the input is 6 bits wide, signed, with 2 fractional bits, and the output is forced to unsigned with 0 fractional bits.  Then an input of -2.0 (1110.00 in binary 2's complement) becomes an output of 56 (111000 in binary)."
      reinterpret3 settings: SourceProductName=The database /home/jmanley/.matlab/R2018a/slblocks_master.db is locked, or a table in the database is locked. (database is locked)
      reinterpret4 settings: SourceProductName=The database /home/jmanley/.matlab/R2018a/slblocks_master.db is locked, or a table in the database is locked. (database is locked)
      reinterpret5 settings: SourceProductName=The database /home/jmanley/.matlab/R2018a/slblocks_master.db is locked, or a table in the database is locked. (database is locked)
      reinterpret6 settings: SourceProductName=The database /home/jmanley/.matlab/R2018a/slblocks_master.db is locked, or a table in the database is locked. (database is locked)
      reinterpret7 settings: SourceProductName=The database /home/jmanley/.matlab/R2018a/slblocks_master.db is locked, or a table in the database is locked. (database is locked)
      reinterpret8 settings: SourceProductName=The database /home/jmanley/.matlab/R2018a/slblocks_master.db is locked, or a table in the database is locked. (database is locked)
      reinterpret9 settings: SourceProductName=The database /home/jmanley/.matlab/R2018a/slblocks_master.db is locked, or a table in the database is locked. (database is locked)
  bus_out : Outport
  wires:
  concatenate/1 -> bus_out/1
  in1/1 -> reinterpret1/1
  reinterpret1/1 -> concatenate/1
  in2/1 -> reinterpret2/1
  reinterpret2/1 -> concatenate/2
  in3/1 -> reinterpret3/1
  reinterpret3/1 -> concatenate/3
  in4/1 -> reinterpret4/1
  reinterpret4/1 -> concatenate/4
  in5/1 -> reinterpret5/1
  reinterpret5/1 -> concatenate/5
  in6/1 -> reinterpret6/1
  reinterpret6/1 -> concatenate/6
  in7/1 -> reinterpret7/1
  reinterpret7/1 -> concatenate/7
  in8/1 -> reinterpret8/1
  reinterpret8/1 -> concatenate/8
  in9/1 -> reinterpret9/1
  reinterpret9/1 -> concatenate/9
  in10/1 -> reinterpret10/1
  reinterpret10/1 -> concatenate/10
  in11/1 -> reinterpret11/1
  reinterpret11/1 -> concatenate/11
  in12/1 -> reinterpret12/1
  reinterpret12/1 -> concatenate/12
  in13/1 -> reinterpret13/1
  reinterpret13/1 -> concatenate/13
  in14/1 -> reinterpret14/1
  reinterpret14/1 -> concatenate/14
  in15/1 -> reinterpret15/1
  reinterpret15/1 -> concatenate/15
  in16/1 -> reinterpret16/1
  reinterpret16/1 -> concatenate/16

== system s_b4a4x32kf_54/sys2/pkt_reord/munge/split ==
  bus_in : Inport
  reinterpret{1..9} (9 alike) : xbsIndex_r4/Reinterpret  force_arith_type=on  arith_type=Unsigned  force_bin_pt=on  bin_pt=0  block_type=reinterpret
      settings: SourceProductName=The database /home/jmanley/.matlab/R2018a/slblocks_master.db is locked, or a table in the database is locked. (database is locked)
  slice1 : xbsIndex_r4/Slice  nbits=32  boolean_output=off  mode=Upper Bit Location + Width  bit1=-225  base1=MSB of Input  bit0=0  base0=LSB of Input  dbl_ovrd=off  block_type=slice
      settings: SourceProductName=The database /home/jmanley/.matlab/R2018a/slblocks_master.db is locked, or a table in the database is locked. (database is locked)
  slice2 : xbsIndex_r4/Slice  nbits=32  boolean_output=off  mode=Upper Bit Location + Width  bit1=-193  base1=MSB of Input  bit0=0  base0=LSB of Input  dbl_ovrd=off  block_type=slice
      settings: SourceProductName=The database /home/jmanley/.matlab/R2018a/slblocks_master.db is locked, or a table in the database is locked. (database is locked)
  slice3 : xbsIndex_r4/Slice  nbits=32  boolean_output=off  mode=Upper Bit Location + Width  bit1=-161  base1=MSB of Input  bit0=0  base0=LSB of Input  dbl_ovrd=off  block_type=slice
      settings: SourceProductName=The database /home/jmanley/.matlab/R2018a/slblocks_master.db is locked, or a table in the database is locked. (database is locked)
  slice4 : xbsIndex_r4/Slice  nbits=32  boolean_output=off  mode=Upper Bit Location + Width  bit1=-129  base1=MSB of Input  bit0=0  base0=LSB of Input  dbl_ovrd=off  block_type=slice
      settings: SourceProductName=The database /home/jmanley/.matlab/R2018a/slblocks_master.db is locked, or a table in the database is locked. (database is locked)
  slice5 : xbsIndex_r4/Slice  nbits=32  boolean_output=off  mode=Upper Bit Location + Width  bit1=-97  base1=MSB of Input  bit0=0  base0=LSB of Input  dbl_ovrd=off  block_type=slice
      settings: SourceProductName=The database /home/jmanley/.matlab/R2018a/slblocks_master.db is locked, or a table in the database is locked. (database is locked)
  slice6 : xbsIndex_r4/Slice  nbits=32  boolean_output=off  mode=Upper Bit Location + Width  bit1=-65  base1=MSB of Input  bit0=0  base0=LSB of Input  dbl_ovrd=off  block_type=slice
      settings: SourceProductName=The database /home/jmanley/.matlab/R2018a/slblocks_master.db is locked, or a table in the database is locked. (database is locked)
  slice7 : xbsIndex_r4/Slice  nbits=32  boolean_output=off  mode=Upper Bit Location + Width  bit1=-33  base1=MSB of Input  bit0=0  base0=LSB of Input  dbl_ovrd=off  block_type=slice
      settings: SourceProductName=The database /home/jmanley/.matlab/R2018a/slblocks_master.db is locked, or a table in the database is locked. (database is locked)
  slice8 : xbsIndex_r4/Slice  nbits=32  boolean_output=off  mode=Upper Bit Location + Width  bit1=-1  base1=MSB of Input  bit0=0  base0=LSB of Input  dbl_ovrd=off  block_type=slice
      settings: SourceProductName=The database /home/jmanley/.matlab/R2018a/slblocks_master.db is locked, or a table in the database is locked. (database is locked)
  slice9 : xbsIndex_r4/Slice  nbits=1  boolean_output=off  mode=Upper Bit Location + Width  bit1=0  base1=MSB of Input  bit0=0  base0=LSB of Input  dbl_ovrd=off  block_type=slice
      settings: SourceProductName=The database /home/jmanley/.matlab/R2018a/slblocks_master.db is locked, or a table in the database is locked. (database is locked)
  msb_out9 : Outport
  out8 : Outport  Port=2
  out7 : Outport  Port=3
  out6 : Outport  Port=4
  out5 : Outport  Port=5
  out4 : Outport  Port=6
  out3 : Outport  Port=7
  out2 : Outport  Port=8
  lsb_out1 : Outport  Port=9
  wires:
  bus_in/1 -> slice9/1, slice8/1, slice7/1, slice6/1, slice5/1, slice4/1, slice3/1, slice2/1, slice1/1
  slice9/1 -> reinterpret9/1
  reinterpret9/1 -> msb_out9/1
  slice8/1 -> reinterpret8/1
  reinterpret8/1 -> out8/1
  slice7/1 -> reinterpret7/1
  reinterpret7/1 -> out7/1
  slice6/1 -> reinterpret6/1
  reinterpret6/1 -> out6/1
  slice5/1 -> reinterpret5/1
  reinterpret5/1 -> out5/1
  slice4/1 -> reinterpret4/1
  reinterpret4/1 -> out4/1
  slice3/1 -> reinterpret3/1
  reinterpret3/1 -> out3/1
  slice2/1 -> reinterpret2/1
  reinterpret2/1 -> out2/1
  slice1/1 -> reinterpret1/1
  reinterpret1/1 -> lsb_out1/1

== system s_b4a4x32kf_54/sys2/pkt_reord/munge1/join ==
  in1 : Inport
  in2 : Inport  Port=2
  concatenate : xbsIndex_r4/Concat  num_inputs=2  dbl_ovrd=off  block_type=concat
      settings: SourceProductName=The database /home/jmanley/.matlab/R2018a/slblocks_master.db is locked, or a table in the database is locked. (database is locked)
  reinterpret1 : xbsIndex_r4/Reinterpret  force_arith_type=on  arith_type=Unsigned  force_bin_pt=on  bin_pt=0  block_type=reinterpret
      settings: SourceProductName=The database /home/jmanley/.matlab/R2018a/slblocks_master.db is locked, or a table in the database is locked. (database is locked)  infoedit="Changes signal type without altering the binary representation.   You can changed the signal between signed and unsigned, and relocate the binary point.<br><br>Hardware notes: In hardware this block costs nothing.<br><br>Example:  Suppose the input is 6 bits wide, signed, with 2 fractional bits, and the output is forced to unsigned with 0 fractional bits.  Then an input of -2.0 (1110.00 in binary 2's complement) becomes an output of 56 (111000 in binary)."
  reinterpret2 : xbsIndex_r4/Reinterpret  force_arith_type=on  arith_type=Unsigned  force_bin_pt=on  bin_pt=0  block_type=reinterpret
      settings: SourceProductName=The database /home/jmanley/.matlab/R2018a/slblocks_master.db is locked, or a table in the database is locked. (database is locked)  infoedit="Changes signal type without altering the binary representation.   You can changed the signal between signed and unsigned, and relocate the binary point.<br><br>Hardware notes: In hardware this block costs nothing.<br><br>Example:  Suppose the input is 6 bits wide, signed, with 2 fractional bits, and the output is forced to unsigned with 0 fractional bits.  Then an input of -2.0 (1110.00 in binary 2's complement) becomes an output of 56 (111000 in binary)."
  bus_out : Outport
  wires:
  concatenate/1 -> bus_out/1
  in1/1 -> reinterpret1/1
  reinterpret1/1 -> concatenate/1
  in2/1 -> reinterpret2/1
  reinterpret2/1 -> concatenate/2
